simulink model "FCSMPC_double_vector_2025b"  (R2025b)
settings: Solver=FixedStepDiscrete  StartTime=0.0  StopTime=2  FixedStep=SimulinkTs  RelTol=1e-3
PreLoadFcn:
  | % Verzeichnis des Modells zum MATLAB-Pfad hinzufügen
  | modelDir = fileparts(get_param(bdroot, 'FileName'));
  | addpath(modelDir);
  | 
  | % Nur der Dateiname – kein Pfad!
  | set_param(bdroot, 'DataDictionary', 'FOC_params.sldd');
model workspace (MAT data in the model file):
  Np : Simulink.Parameter (value not decoded)
values from neighbouring files (symbols this model uses):
  Filter_Current_FilterTimeConst = 3.3333333333333335E-5    [FOC_params.sldd]
  Filter_Current_SensorTimeConst = 1.5915494309189535E-6    [FOC_params.sldd]
  FOC = evalin("base", "FOC")    [createFOC_SLDD.m]
  FOC_Control_Current_KIid = 10.0    [FOC_params.sldd]
  FOC_Control_Current_KIiq = 10.0    [FOC_params.sldd]
  FOC_Control_Current_KPid = 0.20418507462686566    [FOC_params.sldd]
  FOC_Control_Current_KPiq = 0.58674626865671642    [FOC_params.sldd]
  FOC_Control_Current_Krd = 0.8    [FOC_params.sldd]
  FOC_Control_Current_Krq = 0.8    [FOC_params.sldd]
  FOC_Control_Current_TclCur = 0.1    [FOC_params.sldd]
  FOC_Control_Current_Tnd = 0.1    [FOC_params.sldd]
  FOC_Control_Current_Tnq = 0.1    [FOC_params.sldd]
  FOC_Control_InverterVdc_V = 400.0    [FOC_params.sldd]
  FOC_Control_MotorImax_A = 650.0    [FOC_params.sldd]
  FOC_Control_MTPA_MTPV_nT_id_grid = -450.06704889786266 -439.56177000270145 -427.77784873303676 -416.66404703197372 -406.07553272717422 -395.15516533678584 -384.31176061747851 -374.03652088128132 -363.90551910193739 -353.79478643334204 -344.0221683092833 -334.51243453441936 -324.94614350292119 -315.21793409137081 -305.26543360965195 -295.21828280911944 -285.133916324101 -275.01232812136521 -264.86951532374729 -254.7797625148454 -244    [FOC_params.sldd]
  FOC_Control_MTPA_MTPV_nT_iq_grid = -449.09165648258488 -442.56958748923387 -437.25247759546528 -430.91792082419158 -423.83735797306491 -417.11730433547 -410.54064621830616 -403.71584331167304 -396.93611069310379 -390.15794305727007 -382.97216593027133 -375.44639668848538 -367.93447385667577 -360.57088856352266 -353.41289778449368 -346.34020584402072 -339.28416684923008 -332.22010880540631 -325.11927997033376 -317.92299905654966 -31    [FOC_params.sldd]
  FOC_Control_MTPA_MTPV_T_vec = -245.0 -240.0 -235.0 -230.0 -225.0 -220.0 -215.0 -210.0 -205.0 -200.0 -195.0 -190.0 -185.0 -180.0 -175.0 -170.0 -165.0 -160.0 -155.0 -150.0 -145.0 -140.0 -135.0 -130.0 -125.0 -120.0 -115.0 -110.0 -105.0 -100.0 -95.0 -90.0 -85.0 -80.0 -75.0 -70.0 -65.0 -60.0 -55.0 -50.0 -45.0 -40.0 -35.0 -30.0 -25.0 -20.0 -15.0 -10.0 -5.0 0.0 5.0 10.0 15.0 20.0 25.0 30.0 35.0 40.0 45.0 50.0 55.0 60.0 65.0 70.0 75.0    [FOC_params.sldd]
  FOC_Control_MTPA_MTPV_w_vec = 0.0 10.471975511965978 20.943951023931955 31.415926535897931 41.887902047863911 52.359877559829883 62.831853071795862 73.303828583761828 83.775804095727821 94.247779607693786 104.71975511965977 115.19173063162575 125.66370614359172 136.1356816555577 146.60765716752366 157.07963267948966 167.55160819145564 178.02358370342159 188.49555921538757 198.96753472735358 209.43951023931953 219.9114857512855    [FOC_params.sldd]
  FOC_Control_OpenLoop_Id_Ref_A = 0.0    [FOC_params.sldd]
  FOC_Control_OpenLoop_Iq_Ref_A = 0.0    [FOC_params.sldd]
  FOC_Control_OpenLoop_Ud_OpenLoop_V = 0.0    [FOC_params.sldd]
  FOC_Control_OpenLoop_Uq_OpenLoop_V = 0.0    [FOC_params.sldd]
  FOC_Control_RF_omegamech_rad_s = 3141.5926535897934    [FOC_params.sldd]
  FOC_Control_RF_RateCurrent_A = 500.0    [FOC_params.sldd]
  FOC_Control_RF_RateTrq_Nm = 500.0    [FOC_params.sldd]
  FOC_Control_theta_mechOffsetFix = 0.0    [FOC_params.sldd]
  FOC_Control_theta_mechOffsetTime = 0.0    [FOC_params.sldd]
  FOC_Control_TorqueRef_Nm = 10.0    [FOC_params.sldd]
  FOC_Control_Umax_V = 230.94010767585033    [FOC_params.sldd]
  FOC_Flag_ClosedLoopControl = 1.0    [FOC_params.sldd]
  FOC_Flag_ControlStrategy = 2.0    [FOC_params.sldd]
  FOC_Flag_PWMEnable = 1.0    [FOC_params.sldd]
  FOC_Flag_ResetControl = 0.0    [FOC_params.sldd]
  FOC_Flag_TorqueControl = 1.0    [FOC_params.sldd]
  FOC_LUT_DQLimiter_DQ_LUTScaling = 1.8749999999999995E-5    [FOC_params.sldd]
  FOC_PWM_AZSPWMMethod = 3.0    [FOC_params.sldd]
  FOC_PWM_HybridMode = 1.0    [FOC_params.sldd]
  FOC_PWM_LB1 = 0.5    [FOC_params.sldd]
  FOC_PWM_LB2 = 0.77    [FOC_params.sldd]
  FOC_PWM_PWMManuel = 1.0    [FOC_params.sldd]
  FOC_PWM_RSPWMMethod = 2.0    [FOC_params.sldd]
  FOC_PWM_UB1 = 0.66    [FOC_params.sldd]
  FOC_PWM_UB2 = 0.9    [FOC_params.sldd]
  FOC_SampleTime_TsCur = 0.0001    [FOC_params.sldd]
undefined symbols (not defined in the file or in its folder): dspblkCoreblockFVToolHelper, FCS, Filter, gcbh, Plant, SimulinkTs
libraries: hdlsllib x2, simulink x2, autolibfluxpmsm x1
(part 8 of 8)

== matlab function FCSMPC_double_vector_2025b/FCS_MPC/SDA_Solve/SDA Solve/ SDA_Solve_Synchronized ==
  data: H input double size=[15 15]; Jopt output double size=[1 1]; U_unc input double size=[15 1]; NmaxNod input double size=[1 1]; UoptPrev input double size=[15 1]; iabcCompensated input double size=[3 1]; deltaIabcBase input double size=[3 1]; deltaIabcSwitch input double size=[3 3]; lambdaZero input double size=[1 1]; lambdaDeadtime input double size=[1 1]; deadtime_ratio input double size=[1 1]; currentEpsMargin input double size=[1 1]; nodes output double size=[1 1]; optimal output boolean size=[1 1]; Uopt output double size=[15 1]; Uapply output double size=[6 1]; predictionValidNext output boolean size=[1 1]; iabcPredictedNext output double size=[3 1]; leafNodes output double size=[1 1]; bestCMVCost output double size=[1 1]; cmvMetricRatio output double size=[1 1]; switchCountApplied output double size=[1 1]; debug_lower output double size=[3 1]; debug_upper output double size=[3 1]; Jround output double size=[1 1]; Jshift output double size=[1 1]; Jbabai output; solutionToggle output boolean size=[1 1]
function [Jopt, nodes, optimal, Uopt, Uapply, ...
    predictionValidNext,iabcPredictedNext, ...
    leafNodes, bestCMVCost, cmvMetricRatio, switchCountApplied, ...
    debug_lower, debug_upper, Jround, Jshift, Jbabai, solutionToggle] = ...
    SDA_Solve_Synchronized(H, U_unc, NmaxNod, UoptPrev, ...
    iabcCompensated, deltaIabcBase, deltaIabcSwitch, ...
    lambdaZero, lambdaDeadtime, deadtime_ratio, currentEpsMargin)
%SDA_SOLVE Independent double-vector SDA MATLAB Function module.
% The first five ports follow FCSMPC_IdealSDA. Feed Uopt back to UoptPrev
% through a Unit Delay initialized with zeros(15,1). UapplyFirst and
% UapplySecond are applied successively for half an external period each.

Np = 5;
nu = 3;
n = numel(U_unc);

Ubar = H*U_unc;
uprev = UoptPrev(4:6);
deadtimeRatio = deadtime_ratio;

Uround = min(max(round(U_unc),0.0),1.0);
Ushift = zeros(n,1);
Ushift(1:n-nu) = UoptPrev(nu+1:n);
Ushift(n-nu+1:n) = UoptPrev(n-nu+1:n);

% Forward Babai nearest-plane point for the lower-triangular factor H.
% This uses the same conditional centers and binary tie rule as the first
% Schnorr--Euchner descent, but constructs a complete incumbent without
% backtracking.
Ubabai = zeros(n,1);
for babaiLevel = 1:n
    babaiHead = 0.0;
    if babaiLevel > 1
        babaiHead = H(babaiLevel,1:babaiLevel-1)* ...
            Ubabai(1:babaiLevel-1);
    end
    babaiCenter = (Ubar(babaiLevel)-babaiHead)/ ...
        H(babaiLevel,babaiLevel);
    if babaiCenter <= 0.5
        Ubabai(babaiLevel) = 0.0;
    else
        Ubabai(babaiLevel) = 1.0;
    end
end

Jround = norm(H*(Uround-U_unc),2)^2;
Jshift = norm(H*(Ushift-U_unc),2)^2;
Jbabai = norm(H*(Ubabai-U_unc),2)^2;

Uini = Uround;
Jini = Jround;
if Jshift < Jini
    Uini = Ushift;
    Jini = Jshift;
end
if Jbabai < Jini
    Uini = Ubabai;
    Jini = Jbabai;
end

bestCMVCost = sequence_cmv_cost_predicted( ...
    Uini,uprev,iabcCompensated,Np,nu, ...
    deltaIabcBase,deltaIabcSwitch,lambdaZero,lambdaDeadtime, ...
    deadtimeRatio,currentEpsMargin);
bestMetric = Jini+bestCMVCost;
Uopt = Uini;

U = zeros(n,1);
kidx = ones(n,1);
d2s = zeros(n+1,1);
cmvD2s = zeros(n+1,1);
iabcPrediction = zeros(3,Np+1);
iabcPrediction(:,1) = iabcCompensated;
nodes = 0;
leafNodes = 0;
optimal = true;
i = 1;

while i >= 1
    if kidx(i) > 2
        kidx(i) = 1;
        i = i-1;
        continue;
    end
    head = 0.0;
    if i > 1
        head = H(i,1:i-1)*U(1:i-1);
    end
    center = (Ubar(i)-head)/H(i,i);
    if center <= 0.5
        firstCandidate = 0.0;
    else
        firstCandidate = 1.0;
    end
    if kidx(i) == 1
        candidate = firstCandidate;
    else
        candidate = 1.0-firstCandidate;
    end
    kidx(i) = kidx(i)+1;
    U(i) = candidate;
    nodes = nodes+1;
    if NmaxNod > 0 && nodes > NmaxNod
        optimal = false;
        break;
    end

    residual = Ubar(i)-head-H(i,i)*candidate;
    metricNew = d2s(i)+residual*residual;
    cmvMetricNew = cmvD2s(i);
    if mod(i,nu) == 0
        predictionStep = i/nu;
        blockStart = i-nu+1;
        uCurrent = U(blockStart:i);
        if predictionStep == 1
            uPrevious = uprev;
        else
            uPrevious = U(blockStart-nu:blockStart-1);
        end
        iabcBeforeSwitch = iabcPrediction(:,predictionStep);
        [deltaStep,deltaDead] = deadtime_corrected_current_step( ...
            uPrevious,uCurrent,iabcBeforeSwitch, ...
            deltaIabcBase,deltaIabcSwitch,deadtimeRatio,currentEpsMargin);
        cmvIncrement = cmv_cost( ...
            uPrevious,uCurrent,iabcBeforeSwitch,deltaDead, ...
            lambdaZero,lambdaDeadtime,currentEpsMargin);
        metricNew = metricNew+cmvIncrement;
        cmvMetricNew = cmvMetricNew+cmvIncrement;
        iabcPrediction(:,predictionStep+1) = iabcBeforeSwitch+deltaStep;
    end
    if metricNew > bestMetric
        continue;
    end
    if i == n
        leafNodes = leafNodes+1;
        if metricNew < bestMetric
            bestMetric = metricNew;
            Uopt = U;
            bestCMVCost = cmvMetricNew;
        end
    else
        d2s(i+1) = metricNew;
        cmvD2s(i+1) = cmvMetricNew;
        i = i+1;
        kidx(i) = 1;
    end
end

if ~isfinite(bestMetric)
    Uopt = repmat(uprev,Np,1);
end

Uapply = Uopt(1:6);
UapplyFirst = Uopt(1:3);
UapplySecond = Uopt(4:6);

[deltaFirst,~] = deadtime_corrected_current_step( ...
    uprev,UapplyFirst,iabcCompensated, ...
    deltaIabcBase,deltaIabcSwitch, ...
    deadtimeRatio,currentEpsMargin);
iabcAfterFirst = iabcCompensated + deltaFirst;

[deltaSecond,~] = deadtime_corrected_current_step( ...
    UapplyFirst,UapplySecond,iabcAfterFirst, ...
    deltaIabcBase,deltaIabcSwitch,deadtimeRatio,currentEpsMargin);
iabcPredictedNext = iabcAfterFirst+deltaSecond;

switchCountApplied = sum(abs(UapplyFirst-uprev))+ ...
    sum(abs(UapplySecond-UapplyFirst));
Jopt = bestMetric;
if Jopt > eps
    cmvMetricRatio = bestCMVCost/Jopt;
else
    cmvMetricRatio = 0.0;
end
[~,debugDeltaDead] = deadtime_corrected_current_step( ...
    uprev,UapplyFirst,iabcCompensated,deltaIabcBase,deltaIabcSwitch, ...
    deadtimeRatio,currentEpsMargin);
[~,debug_lower,debug_upper] = cmv_cost( ...
    uprev,UapplyFirst,iabcCompensated,debugDeltaDead, ...
    lambdaZero,lambdaDeadtime,currentEpsMargin);
predictionValidNext = true;

% Toggle once after every completed SDA solution. The downstream switch
% detects this edge and explicitly restarts from the first vector.
persistent solutionToggleState
if isempty(solutionToggleState)
    solutionToggleState = false;
end
solutionToggleState = ~solutionToggleState;
solutionToggle = solutionToggleState;
end

function [deltaStep,deltaDead] = deadtime_corrected_current_step( ...
    uPrevious,uCurrent,iabcBeforeSwitch, ...
    deltaBase,deltaSwitch,deadtimeRatio,currentEps)
uDead = uCurrent;
changed = (uPrevious ~= uCurrent);
signEps = 0.1*currentEps;
for phase = 1:3
    if ~changed(phase)
        continue;
    end
    iPhase = iabcBeforeSwitch(phase);
    if iPhase >= signEps
        uDead(phase) = 0.0;
    elseif iPhase <= -signEps
        uDead(phase) = 1.0;
    else
        uDead(phase) = 0.5*(1.0-iPhase/signEps);
    end
end
uEffective = deadtimeRatio*uDead+(1.0-deadtimeRatio)*uCurrent;
deltaDead = deadtimeRatio*(deltaBase+deltaSwitch*uDead);
deltaStep = deltaBase+deltaSwitch*uEffective;
end

function [penalty,lowerBound,upperBound] = cmv_cost( ...
    uPrevious,uCurrent,iabcBeforeSwitch,deltaDead, ...
    lambdaZero,lambdaDeadtime,currentEpsMargin)
penalty = 0.0;
iabcDeadEnd = iabcBeforeSwitch+deltaDead;
lowerBound = min(iabcBeforeSwitch,iabcDeadEnd)-currentEpsMargin;
upperBound = max(iabcBeforeSwitch,iabcDeadEnd)+currentEpsMargin;
uncertain = (lowerBound <= 0.0) & (upperBound >= 0.0);
if all(uCurrent == 0.0) || all(uCurrent == 1.0)
    penalty = penalty+lambdaZero;
end
changed = (uPrevious ~= uCurrent);
if sum(changed) ~= 2
    return;
end
canBeZero = false(3,1);
canBeOne = false(3,1);
for phase = 1:3
    if ~changed(phase)
        canBeZero(phase) = (uPrevious(phase) == 0.0);
        canBeOne(phase) = (uPrevious(phase) == 1.0);
    elseif uncertain(phase)
        canBeZero(phase) = true;
        canBeOne(phase) = true;
    elseif iabcDeadEnd(phase) > 0.0
        canBeZero(phase) = true;
    else
        canBeOne(phase) = true;
    end
end
if all(canBeZero) || all(canBeOne)
    penalty = penalty+lambdaDeadtime;
end
end

function totalPenalty = sequence_cmv_cost_predicted( ...
    U,uprev,iabcInitial,Np,nu,deltaBase,deltaSwitch, ...
    lambdaZero,lambdaDeadtime,deadtimeRatio,currentEpsMargin)
totalPenalty = 0.0;
uPrevious = uprev;
iabcBeforeSwitch = iabcInitial;
for step = 1:Np
    rows = (step-1)*nu+(1:nu);
    uCurrent = U(rows);
    [deltaStep,deltaDead] = deadtime_corrected_current_step( ...
        uPrevious,uCurrent,iabcBeforeSwitch,deltaBase,deltaSwitch, ...
        deadtimeRatio,currentEpsMargin);
    totalPenalty = totalPenalty+cmv_cost( ...
        uPrevious,uCurrent,iabcBeforeSwitch,deltaDead, ...
        lambdaZero,lambdaDeadtime,currentEpsMargin);
    iabcBeforeSwitch = iabcBeforeSwitch+deltaStep;
    uPrevious = uCurrent;
end
end
